simulink model "DC_Pilot_Small"  (R2025a)
settings: Solver=FixedStepDiscrete  StartTime=0.0  StopTime=2  FixedStep=Ts  RelTol=1e-3
undefined symbols (not defined in the file): Ts_relay
libraries: spsSeriesRLCBranchLib x16, spsGroundLib x12, spsDCVoltageSourceLib x2, spsIdealSwitchLib x2, spsCurrentMeasurementLib x2, spsVoltageMeasurementLib x2, sps_lib x1
settings Model: Creator=karth  LastModifiedBy=karth

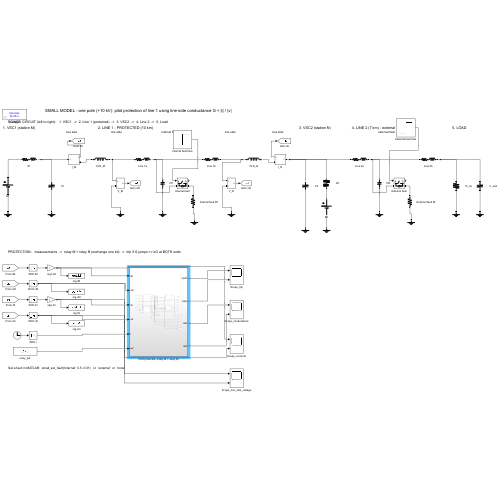
[thumbnail: Simulink's stored preview of the top-level diagram]
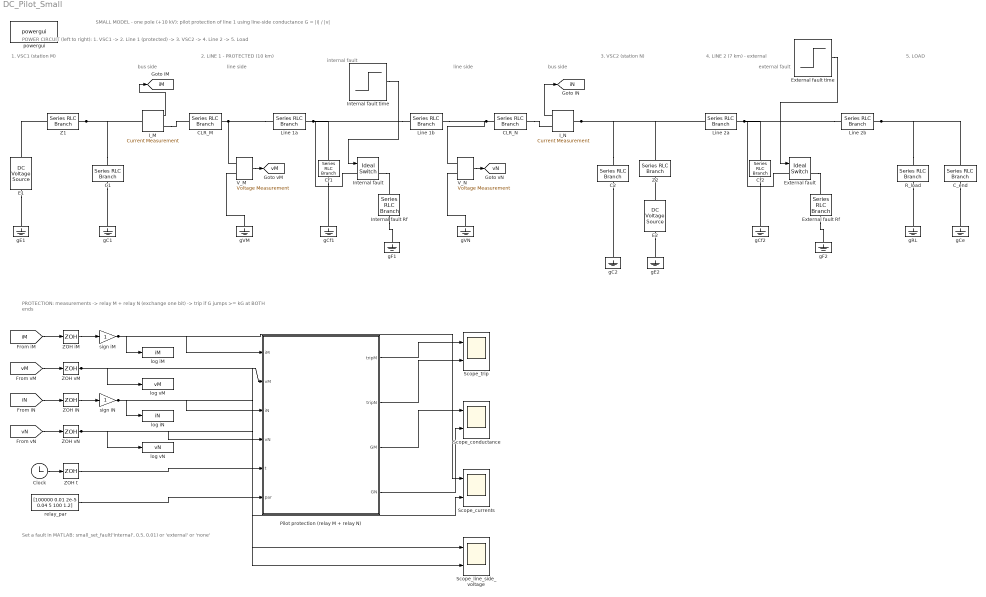
== system DC_Pilot_Small ==
  note: 1. VSC1 (station M)
  note: 2. LINE 1 - PROTECTED (10 km)
  note: 3. VSC2 (station N)
  note: 4. LINE 2 (7 km) - external
  note: 5. LOAD
  note: bus side
  note: line side
  note: internal fault
  note: line side
  note: bus side
  note: external fault
  note: SMALL MODEL - one pole (+10 kV): pilot protection of line 1 using line-side conductance G = |i| / |v|
  note: POWER CIRCUIT (left to right): 1. VSC1 -> 2. Line 1 (protected) -> 3. VSC2 -> 4. Line 2 -> 5. Load
  note: PROTECTION: measurements -> relay M + relay N (exchange one bit) -> trip if G jumps >= kG at BOTH ends
  note: Set a fault in MATLAB: small_set_fault('internal', 0.5, 0.01) or 'external' or 'none'
  C1 : spsSeriesRLCBranchLib/Series RLC Branch  LConnTagsString=__new0  RConnTagsString=__new0  BranchType=C  Resistance=1  Inductance=1e-3  SetiL0=off  InitialCurrent=0  Capacitance=0.5e-3  Setx0=off  InitialVoltage=0  Measurements=None
  C2 : spsSeriesRLCBranchLib/Series RLC Branch  LConnTagsString=__new0  RConnTagsString=__new0  BranchType=C  Resistance=1  Inductance=1e-3  SetiL0=off  InitialCurrent=0  Capacitance=0.5e-3  Setx0=off  InitialVoltage=0  Measurements=None
  CLR_M : spsSeriesRLCBranchLib/Series RLC Branch  LConnTagsString=__new0  RConnTagsString=__new0  BranchType=L  Resistance=1  Inductance=10e-3  SetiL0=off  InitialCurrent=0  Capacitance=1e-6  Setx0=off  InitialVoltage=0  Measurements=None
  CLR_N : spsSeriesRLCBranchLib/Series RLC Branch  LConnTagsString=__new0  RConnTagsString=__new0  BranchType=L  Resistance=1  Inductance=10e-3  SetiL0=off  InitialCurrent=0  Capacitance=1e-6  Setx0=off  InitialVoltage=0  Measurements=None
  C_end : spsSeriesRLCBranchLib/Series RLC Branch  LConnTagsString=__new0  RConnTagsString=__new0  BranchType=C  Resistance=1  Inductance=1e-3  SetiL0=off  InitialCurrent=0  Capacitance=1e-6  Setx0=off  InitialVoltage=0  Measurements=None
  Cf1 : spsSeriesRLCBranchLib/Series RLC Branch  LConnTagsString=__new0  RConnTagsString=__new0  BranchType=C  Resistance=1  Inductance=1e-3  SetiL0=off  InitialCurrent=0  Capacitance=0.2e-6  Setx0=off  InitialVoltage=0  Measurements=None
  Cf2 : spsSeriesRLCBranchLib/Series RLC Branch  LConnTagsString=__new0  RConnTagsString=__new0  BranchType=C  Resistance=1  Inductance=1e-3  SetiL0=off  InitialCurrent=0  Capacitance=0.2e-6  Setx0=off  InitialVoltage=0  Measurements=None
  Clock : Clock
  E1 : spsDCVoltageSourceLib/DC Voltage Source  Amplitude=12900  Measurements=None
  E2 : spsDCVoltageSourceLib/DC Voltage Source  Amplitude=9090  Measurements=None
  External fault : spsIdealSwitchLib/Ideal Switch  Ron=0.001  Lon=0  IC=0  Rs=1e5  Cs=inf  Measurements=on
  External fault Rf : spsSeriesRLCBranchLib/Series RLC Branch  LConnTagsString=__new0  RConnTagsString=__new0  BranchType=R  Resistance=0.01  Inductance=1e-3  SetiL0=off  InitialCurrent=0  Capacitance=1e-6  Setx0=off  InitialVoltage=0  Measurements=None
  External fault time : Step  Time=1000  SampleTime=5e-6
  I_M : spsCurrentMeasurementLib/Current Measurement  PhasorSimulation=off  OutputType=Complex  PSBequivalent=0
  I_N : spsCurrentMeasurementLib/Current Measurement  PhasorSimulation=off  OutputType=Complex  PSBequivalent=0
  Internal fault : spsIdealSwitchLib/Ideal Switch  Ron=0.001  Lon=0  IC=0  Rs=1e5  Cs=inf  Measurements=on
  Internal fault Rf : spsSeriesRLCBranchLib/Series RLC Branch  LConnTagsString=__new0  RConnTagsString=__new0  BranchType=R  Resistance=0.01  Inductance=1e-3  SetiL0=off  InitialCurrent=0  Capacitance=1e-6  Setx0=off  InitialVoltage=0  Measurements=None
  Internal fault time : Step  SampleTime=5e-6
  Line 1a : spsSeriesRLCBranchLib/Series RLC Branch  LConnTagsString=__new0  RConnTagsString=__new0  BranchType=RL  Resistance=0.0695  Inductance=0.795e-3  SetiL0=off  InitialCurrent=0  Capacitance=1e-6  Setx0=off  InitialVoltage=0  Measurements=None
  Line 1b : spsSeriesRLCBranchLib/Series RLC Branch  LConnTagsString=__new0  RConnTagsString=__new0  BranchType=RL  Resistance=0.0695  Inductance=0.795e-3  SetiL0=off  InitialCurrent=0  Capacitance=1e-6  Setx0=off  InitialVoltage=0  Measurements=None
  Line 2a : spsSeriesRLCBranchLib/Series RLC Branch  LConnTagsString=__new0  RConnTagsString=__new0  BranchType=RL  Resistance=0.0487  Inductance=0.557e-3  SetiL0=off  InitialCurrent=0  Capacitance=1e-6  Setx0=off  InitialVoltage=0  Measurements=None
  Line 2b : spsSeriesRLCBranchLib/Series RLC Branch  LConnTagsString=__new0  RConnTagsString=__new0  BranchType=RL  Resistance=0.0487  Inductance=0.557e-3  SetiL0=off  InitialCurrent=0  Capacitance=1e-6  Setx0=off  InitialVoltage=0  Measurements=None
  Pilot protection (relay M + relay N) : Subsystem
  R_load : spsSeriesRLCBranchLib/Series RLC Branch  LConnTagsString=__new0  RConnTagsString=__new0  BranchType=R  Resistance=50  Inductance=1e-3  SetiL0=off  InitialCurrent=0  Capacitance=1e-6  Setx0=off  InitialVoltage=0  Measurements=None
  Scope_conductance : Scope  NumInputPorts=2
      settings: ActiveDisplayYMinimum=-2.5003611990528269  ActiveDisplayYMaximum=22.790912804982568
  Scope_currents : Scope  NumInputPorts=2
      settings: ActiveDisplayYMinimum=-2561.834764167716  ActiveDisplayYMaximum=2562.5634878599467
  Scope_line_side_voltage : Scope  NumInputPorts=2
      settings: ActiveDisplayYMinimum=-4594.9047721845873  ActiveDisplayYMaximum=11641.830345368204
  Scope_trip : Scope  NumInputPorts=2
      settings: ActiveDisplayYMinimum=-0.12499999999999997  ActiveDisplayYMaximum=1.125
  V_M : spsVoltageMeasurementLib/Voltage Measurement  PhasorSimulation=off  OutputType=Complex  PSBequivalent=0
  V_N : spsVoltageMeasurementLib/Voltage Measurement  PhasorSimulation=off  OutputType=Complex  PSBequivalent=0
  Z1 : spsSeriesRLCBranchLib/Series RLC Branch  LConnTagsString=__new0  RConnTagsString=__new0  BranchType=RL  Resistance=10  Inductance=5e-3  SetiL0=off  InitialCurrent=0  Capacitance=1e-6  Setx0=off  InitialVoltage=0  Measurements=None
  Z2 : spsSeriesRLCBranchLib/Series RLC Branch  LConnTagsString=__new0  RConnTagsString=__new0  BranchType=RL  Resistance=10  Inductance=5e-3  SetiL0=off  InitialCurrent=0  Capacitance=1e-6  Setx0=off  InitialVoltage=0  Measurements=None
  ZOH iM : ZeroOrderHold  SampleTime=2e-5
  ZOH iN : ZeroOrderHold  SampleTime=2e-5
  ZOH t : ZeroOrderHold  SampleTime=Ts_relay
  ZOH vM : ZeroOrderHold  SampleTime=2e-5
  ZOH vN : ZeroOrderHold  SampleTime=2e-5
  gC1 : spsGroundLib/Ground  LConnTagsString=a
  gC2 : spsGroundLib/Ground  LConnTagsString=a
  gCe : spsGroundLib/Ground  LConnTagsString=a
  gCf1 : spsGroundLib/Ground  LConnTagsString=a
  gCf2 : spsGroundLib/Ground  LConnTagsString=a
  gE1 : spsGroundLib/Ground  LConnTagsString=a
  gE2 : spsGroundLib/Ground  LConnTagsString=a
  gF1 : spsGroundLib/Ground  LConnTagsString=a
  gF2 : spsGroundLib/Ground  LConnTagsString=a
  gRL : spsGroundLib/Ground  LConnTagsString=a
  gVM : spsGroundLib/Ground  LConnTagsString=a
  gVN : spsGroundLib/Ground  LConnTagsString=a
  log iM : ToWorkspace  VariableName=iM  SaveFormat=Timeseries  SampleTime=-1
  log iN : ToWorkspace  VariableName=iN  SaveFormat=Timeseries  SampleTime=-1
  log vM : ToWorkspace  VariableName=vM  SaveFormat=Timeseries  SampleTime=-1
  log vN : ToWorkspace  VariableName=vN  SaveFormat=Timeseries  SampleTime=-1
  powergui : sps_lib/powergui  Priority=1  SimulationMode=Discrete  SampleTime=5e-06  frequency=60  Iterations=50  frequencyindice=0  Pbase=100e6  ErrMax=1e-4  UnitsV=kV  UnitsW=MW  buscounter=0  FunctionMessages=off  echomessages=off  EnableUseOfTLC=off  CurrentSourceSwitches=off  DisableSnubberDevices=off  DisableRonSwitches=off  DisableVfSwitches=off  DisplayEquations=off  AutomaticDiscreteSolvers=off  SolverType=Tustin/Backward Euler (TBE)  Interpol=off  ExternalGateDelay=off  methode=off  Ts=100  x0status=blocks  SPID=on  SwTol=0  HookPort=off  NonlinearTolerance=1e-4  nMaxIteration=100  ContinueOnMaxIteration=off  RestoreLinks=warning  ResistiveCurrentMeasurement=off  Frange=[0:2:500]  Ylog=off  Xlog=on  ShowGrid=off  save=off  variable=ZData  structure=0  ZoomFFT=off  StartTime=0.0  cycles=1  DisplayStyle=1  fundamental=60  FreqAxis=off  MaxFrequency=1000  frequencyindicesteady=1  RmsSteady=1  display=off
  relay_par : Constant  Value="[100000  0.01  2e-5  0.04  5  100  1.2]"
  sign iM : Gain
  sign iN : Gain
  tag scope: iM=global, iN=global, vM=global, vN=global
  wires:
  Internal fault time/1 -> Internal fault/1
  I_M/1 -> [iM]
  I_N/1 -> [iN]
  V_M/1 -> [vM]
  V_N/1 -> [vN]
  External fault time/1 -> External fault/1
  [iM] -> ZOH iM/1
  ZOH iM/1 -> sign iM/1
  sign iM/1 -> log iM/1, Pilot protection (relay M + relay N)/1(iM), Scope_currents/1
  [vM] -> ZOH vM/1
  ZOH vM/1 -> log vM/1, Pilot protection (relay M + relay N)/2(vM), Scope_line_side_voltage/1
  [iN] -> ZOH iN/1
  ZOH iN/1 -> sign iN/1
  sign iN/1 -> log iN/1, Pilot protection (relay M + relay N)/3(iN), Scope_currents/2
  [vN] -> ZOH vN/1
  ZOH vN/1 -> log vN/1, Pilot protection (relay M + relay N)/4(vN), Scope_line_side_voltage/2
  Clock/1 -> ZOH t/1
  ZOH t/1 -> Pilot protection (relay M + relay N)/5(t)
  relay_par/1 -> Pilot protection (relay M + relay N)/6(par)
  Pilot protection (relay M + relay N)/1(tripM) -> Scope_trip/1
  Pilot protection (relay M + relay N)/2(tripN) -> Scope_trip/2
  Pilot protection (relay M + relay N)/3(GM) -> Scope_conductance/1
  Pilot protection (relay M + relay N)/4(GN) -> Scope_conductance/2
  connections:
  C1/LConn1 -- Z1/RConn1 -- I_M/LConn1
  C1/RConn1 -- gC1/LConn1
  I_M/RConn1 -- CLR_M/LConn1
  Line 1a/LConn1 -- CLR_M/RConn1 -- V_M/LConn1
  Line 1b/LConn1 -- Line 1a/RConn1 -- Cf1/LConn1 -- Internal fault/LConn1
  CLR_N/LConn1 -- Line 1b/RConn1 -- V_N/LConn1
  CLR_N/RConn1 -- I_N/RConn1
  V_M/LConn2 -- gVM/LConn1
  V_N/LConn2 -- gVN/LConn1
  Cf1/RConn1 -- gCf1/LConn1
  Internal fault/RConn1 -- Internal fault Rf/LConn1
  Internal fault Rf/RConn1 -- gF1/LConn1
  C2/LConn1 -- I_N/LConn1 -- Z2/LConn1 -- Line 2a/LConn1
  C2/RConn1 -- gC2/LConn1
  Line 2b/LConn1 -- Line 2a/RConn1 -- Cf2/LConn1 -- External fault/LConn1
  Cf2/RConn1 -- gCf2/LConn1
  External fault/RConn1 -- External fault Rf/LConn1
  External fault Rf/RConn1 -- gF2/LConn1
  R_load/LConn1 -- Line 2b/RConn1 -- C_end/LConn1
  R_load/RConn1 -- gRL/LConn1
  C_end/RConn1 -- gCe/LConn1
  E2/RConn1 -- Z2/RConn1
  E2/LConn1 -- gE2/LConn1
  E1/RConn1 -- Z1/LConn1
  E1/LConn1 -- gE1/LConn1

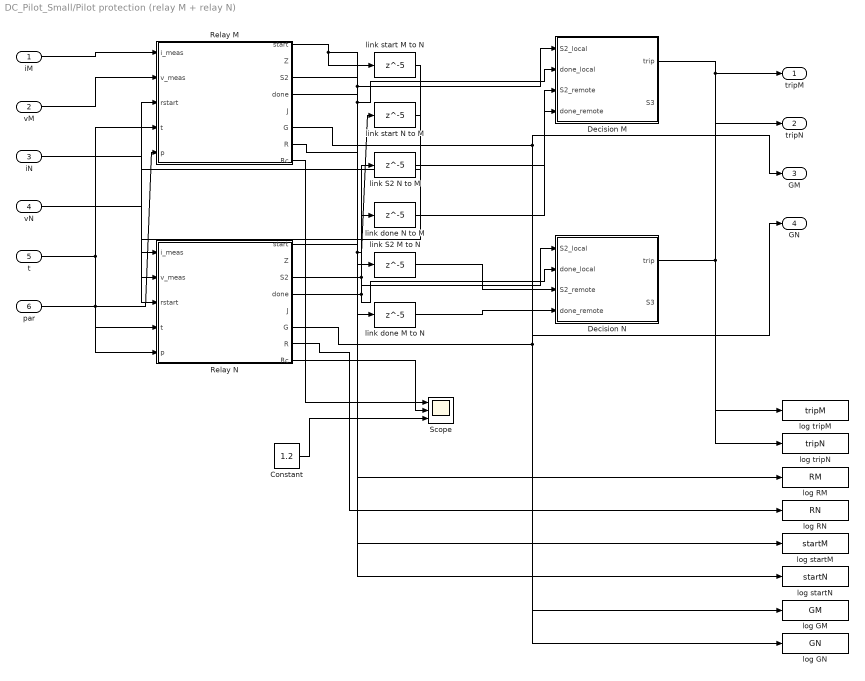
== system DC_Pilot_Small/Pilot protection (relay M + relay N) ==
  iM : Inport
  vM : Inport  Port=2
  iN : Inport  Port=3
  vN : Inport  Port=4
  t : Inport  Port=5
  par : Inport  Port=6
  Constant : Constant  Value=1.2
  Decision M : MATLAB Function  TreatAsAtomicUnit=on
  Decision N : MATLAB Function  TreatAsAtomicUnit=on
  Relay M : MATLAB Function  TreatAsAtomicUnit=on
  Relay N : MATLAB Function  TreatAsAtomicUnit=on
  Scope : Scope  NumInputPorts=3
      settings: ActiveDisplayYMinimum=-2.1653733474042649E+9  ActiveDisplayYMaximum=1.948836013663839E+10
  link S2 M to N : Delay  DelayLength=5  InitialCondition=0  SampleTime=2e-5
  link S2 N to M : Delay  DelayLength=5  InitialCondition=0  SampleTime=2e-5
  link done M to N : Delay  DelayLength=5  InitialCondition=0  SampleTime=2e-5
  link done N to M : Delay  DelayLength=5  InitialCondition=0  SampleTime=2e-5
  link start M to N : Delay  DelayLength=5  InitialCondition=0  SampleTime=2e-5
  link start N to M : Delay  DelayLength=5  InitialCondition=0  SampleTime=2e-5
  log GM : ToWorkspace  VariableName=GM  SaveFormat=Timeseries  SampleTime=-1
  log GN : ToWorkspace  VariableName=GN  SaveFormat=Timeseries  SampleTime=-1
  log RM : ToWorkspace  VariableName=RM  SaveFormat=Timeseries  SampleTime=-1
  log RN : ToWorkspace  VariableName=RN  SaveFormat=Timeseries  SampleTime=-1
  log startM : ToWorkspace  VariableName=startM  SaveFormat=Timeseries  SampleTime=-1
  log startN : ToWorkspace  VariableName=startN  SaveFormat=Timeseries  SampleTime=-1
  log tripM : ToWorkspace  VariableName=tripM  SaveFormat=Timeseries  SampleTime=-1
  log tripN : ToWorkspace  VariableName=tripN  SaveFormat=Timeseries  SampleTime=-1
  tripM : Outport
  tripN : Outport  Port=2
  GM : Outport  Port=3
  GN : Outport  Port=4
  wires:
  iM/1 -> Relay M/1(i_meas)
  vM/1 -> Relay M/2(v_meas)
  t/1 -> Relay M/4(t), Relay N/4(t)
  par/1 -> Relay M/5(p), Relay N/5(p)
  iN/1 -> Relay N/1(i_meas)
  vN/1 -> Relay N/2(v_meas)
  Relay M/1(start) -> link start M to N/1, log startM/1
  link start M to N/1 -> Relay N/3(rstart)
  Relay N/1(start) -> link start N to M/1, log startN/1
  link start N to M/1 -> Relay M/3(rstart)
  Relay N/3(S2) -> Decision N/1(S2_local), link S2 N to M/1
  link S2 N to M/1 -> Decision M/3(S2_remote)
  Relay N/4(done) -> Decision N/2(done_local), link done N to M/1
  link done N to M/1 -> Decision M/4(done_remote)
  Relay M/3(S2) -> link S2 M to N/1, Decision M/1(S2_local)
  link S2 M to N/1 -> Decision N/3(S2_remote)
  Relay M/4(done) -> link done M to N/1, Decision M/2(done_local)
  link done M to N/1 -> Decision N/4(done_remote)
  Decision M/1(trip) -> tripM/1, log tripM/1
  Decision N/1(trip) -> tripN/1, log tripN/1
  Relay M/6(G) -> GM/1, log GM/1
  Relay N/6(G) -> GN/1, log GN/1
  Relay M/7(R) -> log RM/1
  Relay N/7(R) -> log RN/1
  Constant/1 -> Scope/3
  Relay N/8(Rc) -> Scope/2
  Relay M/8(Rc) -> Scope/1

== matlab function DC_Pilot_Small/Pilot protection (relay M + relay N)/Relay N ==
  data: i_meas input; start output; v_meas input; rstart input; t input; p input; Z output; S2 output; done output; J output; G output; R output; Rc output
function [start, Z, S2, done, J, G, R, Rc] = pilot_relay_newrule(i_meas, v_meas, rstart, t, p)
%#codegen
% One end of the integral-increment pilot protection (Li et al., IEEE TSG 2026)
% with CONDUCTANCE G = |i|/|v| (line-side voltage) and a NEW local criterion:
%   R  = mean G in the first 0.1 ms after start / mean G in the 0.5 ms before start
%   S2 = 1 if R >= kG  ("this end saw a conductance jump")
% For an internal fault the line-side voltage collapses at BOTH ends (both meters are
% between the two CLRs, on the faulted side), so both ends report S2 = 1.
% For an external fault the line-side voltages hardly move, so R stays ~1.
%   i_meas : line current at this end (A)
%   v_meas : pole-to-ground voltage at this relay's measuring point (V)
%   rstart : start signal from the other end (after the comm delay)
%   t      : time (s)
%   p      : [k1 k2 Ts t_en cd vmin kG]
% Outputs: start, Z (paper's integral criterion, for reference), S2 (1 = jump >= kG), done,
%          J(T) for T = 0..0.5 ms, G (S), R (jump ratio)

Nbuf = 250;          % data cache: 5 ms at 50 kHz
Nw   = 25;           % 0.5 ms data window
Nsmf = 5;            % sliding mean filter, 0.1 ms

persistent ibuf gbuf fbuf cnt started s0 Zs S2s dn Js Rs refHold
if isempty(ibuf)
    ibuf = zeros(Nbuf,1); gbuf = zeros(Nbuf,1); fbuf = zeros(Nbuf,1);
    cnt = 0; started = false; s0 = 0;
    Zs = 0; S2s = 0; dn = false; Js = zeros(Nw+1,1); Rs = 1;
        refHold = 0;
end

k1 = p(1); k2 = p(2); Ts = p(3); t_en = p(4); cd = min(max(p(5),0), Nbuf-2*Nw); vmin = p(6); kG = p(7);

% ---- conductance
g = abs(i_meas)/max(abs(v_meas), vmin);

% ---- data cache + sliding mean filter (Eq. 18)
cnt = cnt + 1;
ibuf(1:Nbuf-1) = ibuf(2:Nbuf); ibuf(Nbuf) = i_meas;
gbuf(1:Nbuf-1) = gbuf(2:Nbuf); gbuf(Nbuf) = g;
fbuf(1:Nbuf-1) = fbuf(2:Nbuf); fbuf(Nbuf) = sum(gbuf(Nbuf-Nsmf+1:Nbuf))/Nsmf;

% ---- start criterion on the current (Eqs. 10-11), as in the paper
didt = (3*ibuf(Nbuf-4) - 16*ibuf(Nbuf-3) + 36*ibuf(Nbuf-2) - 48*ibuf(Nbuf-1) + 25*ibuf(Nbuf))/(12*Ts);
if ~started && t >= t_en && cnt > Nbuf
    if abs(didt) > k1
        started = true; s0 = cnt;
    elseif rstart > 0.5
        started = true; s0 = cnt - cd;
    end
    if started
        k0 = Nbuf - (cnt - s0);
        refHold = max(sum(fbuf(k0-5:k0-1))/5, 1e-12);   % mean G in 0.1 ms before start
    end
end

% ---- integral increment of G (Eqs. 7, 13) and criterion Z (Eqs. 12, 14, 15)
if started && ~dn && cnt >= s0 + Nw
    idx0 = Nbuf - (cnt - s0);
   ref = 0;
for k = idx0-5 : idx0-1
    ref = ref + fbuf(k);
end
ref = max(ref/5, 1e-12);
    area = 0;
    for n = 1:Nw
        area = area + Ts*(fbuf(idx0+n-1) + fbuf(idx0+n))/2;
        Js(n+1) = area/(ref*n*Ts) - 1;
    end
    Zs = (Ts*1e3)*(sum(Js) - 0.5*(Js(1) + Js(Nw+1)));
    % NEW criterion: conductance jump in the first 0.1 ms (5 samples)
    early = 0;
    for k = idx0+1 : idx0+5
        early = early + fbuf(k);
    end
    Rs = (early/5)/ref;
    if Rs >= kG
        S2s = 1;
    else
        S2s = 0;
    end
    dn = true;
end
% ---- continuous conductance jump ratio (for display only)
now5 = sum(fbuf(Nbuf-4:Nbuf))/5;                         % mean G of latest 0.1 ms
if cnt <= Nbuf || t < t_en
    Rc = 1;                                              % buffer not full yet
elseif started
    Rc = now5/refHold;                                   % compared with G before the start
else
    Rc = now5/max(sum(fbuf(Nbuf-9:Nbuf-5))/5, 1e-6);     % ~1 in normal operation
end

start = double(started);
Z     = Zs;
S2    = S2s;
done  = double(dn);
J     = Js;
G     = g;
R     = Rs;
end

== matlab function DC_Pilot_Small/Pilot protection (relay M + relay N)/Relay M ==
  data: i_meas input; start output; v_meas input; rstart input; t input; p input; Z output; S2 output; done output; J output; G output; R output; Rc output
function [start, Z, S2, done, J, G, R, Rc] = pilot_relay_newrule(i_meas, v_meas, rstart, t, p)
%#codegen
% One end of the integral-increment pilot protection (Li et al., IEEE TSG 2026)
% with CONDUCTANCE G = |i|/|v| (line-side voltage) and a NEW local criterion:
%   R  = mean G in the first 0.1 ms after start / mean G in the 0.5 ms before start
%   S2 = 1 if R >= kG  ("this end saw a conductance jump")
% For an internal fault the line-side voltage collapses at BOTH ends (both meters are
% between the two CLRs, on the faulted side), so both ends report S2 = 1.
% For an external fault the line-side voltages hardly move, so R stays ~1.
%   i_meas : line current at this end (A)
%   v_meas : pole-to-ground voltage at this relay's measuring point (V)
%   rstart : start signal from the other end (after the comm delay)
%   t      : time (s)
%   p      : [k1 k2 Ts t_en cd vmin kG]
% Outputs: start, Z (paper's integral criterion, for reference), S2 (1 = jump >= kG), done,
%          J(T) for T = 0..0.5 ms, G (S), R (jump ratio)

Nbuf = 250;          % data cache: 5 ms at 50 kHz
Nw   = 25;           % 0.5 ms data window
Nsmf = 5;            % sliding mean filter, 0.1 ms

persistent ibuf gbuf fbuf cnt started s0 Zs S2s dn Js Rs refHold
if isempty(ibuf)
    ibuf = zeros(Nbuf,1); gbuf = zeros(Nbuf,1); fbuf = zeros(Nbuf,1);
    cnt = 0; started = false; s0 = 0;
    Zs = 0; S2s = 0; dn = false; Js = zeros(Nw+1,1); Rs = 1;
        refHold = 0;
end

k1 = p(1); k2 = p(2); Ts = p(3); t_en = p(4); cd = min(max(p(5),0), Nbuf-2*Nw); vmin = p(6); kG = p(7);

% ---- conductance
g = abs(i_meas)/max(abs(v_meas), vmin);

% ---- data cache + sliding mean filter (Eq. 18)
cnt = cnt + 1;
ibuf(1:Nbuf-1) = ibuf(2:Nbuf); ibuf(Nbuf) = i_meas;
gbuf(1:Nbuf-1) = gbuf(2:Nbuf); gbuf(Nbuf) = g;
fbuf(1:Nbuf-1) = fbuf(2:Nbuf); fbuf(Nbuf) = sum(gbuf(Nbuf-Nsmf+1:Nbuf))/Nsmf;

% ---- start criterion on the current (Eqs. 10-11), as in the paper
didt = (3*ibuf(Nbuf-4) - 16*ibuf(Nbuf-3) + 36*ibuf(Nbuf-2) - 48*ibuf(Nbuf-1) + 25*ibuf(Nbuf))/(12*Ts);
if ~started && t >= t_en && cnt > Nbuf
    if abs(didt) > k1
        started = true; s0 = cnt;
    elseif rstart > 0.5
        started = true; s0 = cnt - cd;
    end
    if started
        k0 = Nbuf - (cnt - s0);
        refHold = max(sum(fbuf(k0-5:k0-1))/5, 1e-12);   % mean G in 0.1 ms before start
    end
end
% ---- integral increment of G (Eqs. 7, 13) and criterion Z (Eqs. 12, 14, 15)
if started && ~dn && cnt >= s0 + Nw
    idx0 = Nbuf - (cnt - s0);
   ref = 0;
for k = idx0-5 : idx0-1
    ref = ref + fbuf(k);
end
ref = max(ref/5, 1e-12);
    area = 0;
    for n = 1:Nw
        area = area + Ts*(fbuf(idx0+n-1) + fbuf(idx0+n))/2;
        Js(n+1) = area/(ref*n*Ts) - 1;
    end
    Zs = (Ts*1e3)*(sum(Js) - 0.5*(Js(1) + Js(Nw+1)));
    % NEW criterion: conductance jump in the first 0.1 ms (5 samples)
    early = 0;
    for k = idx0+1 : idx0+5
        early = early + fbuf(k);
    end
    Rs = (early/5)/ref;
    if Rs >= kG
        S2s = 1;
    else
        S2s = 0;
    end
    dn = true;
end
% ---- continuous conductance jump ratio (for display only)
now5 = sum(fbuf(Nbuf-4:Nbuf))/5;                         % mean G of latest 0.1 ms
if cnt <= Nbuf || t < t_en
    Rc = 1;                                              % buffer not full yet
elseif started
    Rc = now5/refHold;                                   % compared with G before the start
else
    Rc = now5/max(sum(fbuf(Nbuf-9:Nbuf-5))/5, 1e-6);     % ~1 in normal operation
end

start = double(started);
Z     = Zs;
S2    = S2s;
done  = double(dn);
J     = Js;
G     = g;
R     = Rs;
end

== matlab function DC_Pilot_Small/Pilot protection (relay M + relay N)/Decision M ==
  data: S2_local input; trip output; done_local input; S2_remote input; done_remote input; S3 output
function [trip, S3] = pilot_decision_and(S2_local, done_local, S2_remote, done_remote)
%#codegen
% NEW fault identification for line-side conductance:
% internal fault (trip) only if BOTH ends saw a conductance jump (S2 = 1 at M AND at N).
% Only one logical bit per end is exchanged, as in the paper's pilot scheme.
persistent latched
if isempty(latched), latched = false; end
S3 = 1;
if done_local > 0.5 && done_remote > 0.5
    if S2_local > 0.5 && S2_remote > 0.5
        S3 = 0;
        latched = true;
    end
end
trip = double(latched);
end

== matlab function DC_Pilot_Small/Pilot protection (relay M + relay N)/Decision N ==
  data: S2_local input; trip output; done_local input; S2_remote input; done_remote input; S3 output
function [trip, S3] = pilot_decision_and(S2_local, done_local, S2_remote, done_remote)
%#codegen
% NEW fault identification for line-side conductance:
% internal fault (trip) only if BOTH ends saw a conductance jump (S2 = 1 at M AND at N).
% Only one logical bit per end is exchanged, as in the paper's pilot scheme.
persistent latched
if isempty(latched), latched = false; end
S3 = 1;
if done_local > 0.5 && done_remote > 0.5
    if S2_local > 0.5 && S2_remote > 0.5
        S3 = 0;
        latched = true;
    end
end
trip = double(latched);
end
